simulink model "MMC_Per_arm_outer_v5_G2_case2_clip_delay1p4_aligned"  (R2024a)
settings: Solver=FixedStepDiscrete  StartTime=0.0  StopTime=2  FixedStep=Ts  RelTol=1e-3
PreLoadFcn:
  | % ---- MMC_Inner4 workspace parameters (control gains live inside the MATLAB Function blocks) ----
  | % ---------------- Converter ----------------
  | VDC     = 800;                  % DC-link voltage (V)  -> Vdc_pos / Vdc_neg = VDC/2
  | N       = 8;                    % submodules per arm
  | C       = 2.2e-3;               % submodule capacitance (F)  -> HB_xx blocks
  | vo      = 100;                  % nominal = initial capacitor voltage (V) = VDC/N  -> HB_xx, Vc_nom
  | W_nom   = 0.5*C*N*vo^2;         % nominal arm energy (J) -> initial condition of the Comm delay blocks
  | Larm    = 5e-3;                 % arm inductance (H)
  | Rarm    = 0.5;                  % arm resistance (ohm)
  | 
  | % ---------------- Grid and PCC filter ----------------
  | f       = 50;                   % grid frequency (Hz)
  | Vg_rms  = 230;                  % grid RMS voltage (V)
  | Vg_pk   = Vg_rms*sqrt(2);       % grid peak voltage (V) -> AC Voltage Source
  | Lg      = 2e-3;                 % line inductance (H)
  | Rg      = 0.1;                  % line resistance (ohm)
  | Cf      = 10e-6;                % AC filter capacitance (F)
  | Rf      = 10;                   % AC filter damping resistance (ohm)
  | 
  | % ---------------- Power set-points ----------------
  | Pstar   = 1500;                 % active-power set-point (W)
  | Qstar   = 0;                    % reactive-power set-point (var)
  | 
  | % ---------------- Timing ----------------
  | fsw     = 1250;                 % carrier frequency per submodule (Hz) -> N*fsw = 10 kHz per arm
  | Ts      = 1e-5;                 % simulation step = submodule-layer step (s)
  | Ts_ctrl = 1e-4;                 % arm-leader control step (s)
  | % ---------------- Test schedule: P* staircase and PCC load (added in _tests) ----------------
  | P_base   = 1500;                % staircase base = first level (W)
  | dP_step  = 250;                 % staircase step (W): 1500 -> 1750 -> 2000 -> 2250 -> 2500
  | t_step   = [0.6 1.0 1.4 1.8];   % step instants (s), 0.4 s hold at each level
  | t_back   = 2.2;                 % return to P_base (s) before the load test
  | P_load1  = 1000;                % PCC load 1 (W at 230 V rms)
  | P_load2  = 1000;                % PCC load 2 (W at 230 V rms)
  | R_load1  = Vg_rms^2/P_load1;    % 52.9 ohm
  | R_load2  = Vg_rms^2/P_load2;    % 52.9 ohm
  | t_load1  = 2.4;                 % Breaker load 1: closes at 2.4 s (stays closed)
  | t_load2  = [2.7 3.0];           % Breaker load 2: closes at 2.7 s, opens at 3.0 s
  | % ---- CASE: initial imbalance HB_u3 = 110 V, HB_u6 = 90 V, P* fixed 1500 W, no PCC load, 2 s
  | % ---- DERIVED: case2_clip_delay1p4_aligned: case 2 clip + time-aligned delay 140 samples (1.4 ms) -- eq. (6) test below the bound
  | % ---- DERIVED: case2_clip: same as case 2 + correction bounded to |k_v*err| <= 0.1 in hb_sm_local_ctrl (16 charts)
  | % P_SLEW = 5000 W/s, I_max = 17 A, P_max = 2500 W are set INSIDE mmc_outer_ctrl (both arm leaders)
  | t_load1  = 10;  t_load2 = [10 11];   % PCC load test disabled in this case (beyond StopTime)
  | Vc0_u3   = 110;                 % initial capacitor voltage of HB_u3 (V)
  | Vc0_u6   = 90;                  % initial capacitor voltage of HB_u6 (V)
InitFcn:
  | % ---- MMC_Inner4 workspace parameters (control gains live inside the MATLAB Function blocks) ----
  | % ---------------- Converter ----------------
  | VDC     = 800;                  % DC-link voltage (V)  -> Vdc_pos / Vdc_neg = VDC/2
  | N       = 8;                    % submodules per arm
  | C       = 2.2e-3;               % submodule capacitance (F)  -> HB_xx blocks
  | vo      = 100;                  % nominal = initial capacitor voltage (V) = VDC/N  -> HB_xx, Vc_nom
  | W_nom   = 0.5*C*N*vo^2;         % nominal arm energy (J) -> initial condition of the Comm delay blocks
  | Larm    = 5e-3;                 % arm inductance (H)
  | Rarm    = 0.5;                  % arm resistance (ohm)
  | 
  | % ---------------- Grid and PCC filter ----------------
  | f       = 50;                   % grid frequency (Hz)
  | Vg_rms  = 230;                  % grid RMS voltage (V)
  | Vg_pk   = Vg_rms*sqrt(2);       % grid peak voltage (V) -> AC Voltage Source
  | Lg      = 2e-3;                 % line inductance (H)
  | Rg      = 0.1;                  % line resistance (ohm)
  | Cf      = 10e-6;                % AC filter capacitance (F)
  | Rf      = 10;                   % AC filter damping resistance (ohm)
  | 
  | % ---------------- Power set-points ----------------
  | Pstar   = 1500;                 % active-power set-point (W)
  | Qstar   = 0;                    % reactive-power set-point (var)
  | 
  | % ---------------- Timing ----------------
  | fsw     = 1250;                 % carrier frequency per submodule (Hz) -> N*fsw = 10 kHz per arm
  | Ts      = 1e-5;                 % simulation step = submodule-layer step (s)
  | Ts_ctrl = 1e-4;                 % arm-leader control step (s)
  | % ---------------- Test schedule: P* staircase and PCC load (added in _tests) ----------------
  | P_base   = 1500;                % staircase base = first level (W)
  | dP_step  = 250;                 % staircase step (W): 1500 -> 1750 -> 2000 -> 2250 -> 2500
  | t_step   = [0.6 1.0 1.4 1.8];   % step instants (s), 0.4 s hold at each level
  | t_back   = 2.2;                 % return to P_base (s) before the load test
  | P_load1  = 1000;                % PCC load 1 (W at 230 V rms)
  | P_load2  = 1000;                % PCC load 2 (W at 230 V rms)
  | R_load1  = Vg_rms^2/P_load1;    % 52.9 ohm
  | R_load2  = Vg_rms^2/P_load2;    % 52.9 ohm
  | t_load1  = 2.4;                 % Breaker load 1: closes at 2.4 s (stays closed)
  | t_load2  = [2.7 3.0];           % Breaker load 2: closes at 2.7 s, opens at 3.0 s
  | % ---- CASE: initial imbalance HB_u3 = 110 V, HB_u6 = 90 V, P* fixed 1500 W, no PCC load, 2 s
  | % ---- DERIVED: case2_clip_delay1p4_aligned: case 2 clip + time-aligned delay 140 samples (1.4 ms) -- eq. (6) test below the bound
  | % ---- DERIVED: case2_clip: same as case 2 + correction bounded to |k_v*err| <= 0.1 in hb_sm_local_ctrl (16 charts)
  | % P_SLEW = 5000 W/s, I_max = 17 A, P_max = 2500 W are set INSIDE mmc_outer_ctrl (both arm leaders)
  | t_load1  = 10;  t_load2 = [10 11];   % PCC load test disabled in this case (beyond StopTime)
  | Vc0_u3   = 110;                 % initial capacitor voltage of HB_u3 (V)
  | Vc0_u6   = 90;                  % initial capacitor voltage of HB_u6 (V)
libraries: spsHalfBridgeMMCLib x16, spsSeriesRLCBranchLib x6, spsCurrentMeasurementLib x5, spsBreakerLib x2, spsGroundLib x2, spsDCVoltageSourceLib x2, spsACVoltageSourceLib x1, spspowerguiLib x1, spsVoltageMeasurementLib x1
(part 4 of 6)

== matlab function MMC_Per_arm_outer_v5_G2_case2_clip_delay1p4_aligned/SM_l7/Local Ctrl ==
  data: sm_id input; S_top output; m_arm input; i_arm input; Vc_i input; Vc_prev input; Vc_next input; t input; S_bot output
function [S_top, S_bot] = hb_sm_local_ctrl(sm_id, m_arm, i_arm, Vc_i, Vc_prev, Vc_next, t)
%#codegen
% =========================================================================
% HB_SM_LOCAL_CTRL  -  Submodule local controller: neighbour balancing + PSC-PWM
% -------------------------------------------------------------------------
% Block     : "Local Ctrl" inside every SM_ux / SM_lx subsystem
% Rate      : Ts = 10 us
% Instances : 16 (one per half-bridge submodule)
% Purpose   : decide the two gate signals of ONE half-bridge submodule using
%             only local information: own capacitor voltage, the two ring
%             neighbours, the arm modulation index sent by the arm leader,
%             the arm-current direction and the time base.
%             No sorting and no access to the full capacitor-voltage vector.
% Inputs    : sm_id    own index 1..N (sets the carrier phase shift)
%             m_arm    arm modulation index from the arm leader, in [0, 1]
%             i_arm    arm current (A), only its direction is used
%             Vc_i     own capacitor voltage (V)
%             Vc_prev  previous ring neighbour voltage (V)
%             Vc_next  next ring neighbour voltage (V)
%             t        simulation time (s), carrier time base
% Outputs   : S_top    upper switch gate (1 = on)  -> capacitor INSERTED (+Vc)
%             S_bot    lower switch gate (1 = on)  -> capacitor BYPASSED (0 V)
% =========================================================================

%% ---------------- PARAMETERS ----------------
N      = 8;                              % submodules per arm -> carrier phase shift of SM k = (k-1)/N of a period
fsw    = 1250;                           % carrier frequency per submodule (Hz) -> N*fsw = 10 kHz apparent arm ripple
k_v    = 0.2;                            % balancing gain (1/V): modulation-index change per volt of error
dead   = 0.1;                            % dead-band (V): errors smaller than this are ignored (no chattering)
Iscale = 1.0;                            % current scale (A) of the smooth sign function tanh(i_arm/Iscale)
dm_max = 0.1;                            % BOUND on the correction: |k_v*err| <= dm_max  (CLIP case, Delta d_max = 0.1)

%% ---------------- 1. neighbour-average balancing correction ----------------
err  = 0.5*(Vc_prev + Vc_next) - Vc_i;   % error = neighbour average - own voltage (> 0: I am too low, I need charging)
if abs(err) < dead                       % error inside the dead-band?
    err = 0;                             % ignore it
end
dirn = tanh(i_arm / Iscale);             % smooth current direction in (-1, +1); > 0 means inserting CHARGES the capacitor
c    = min(max(k_v * err, -dm_max), dm_max);   % bounded correction magnitude: |k_v e_i| <= dm_max (a 10 V error no longer saturates the duty)
dm   = c * dirn;                         % correction: insert more if charging is needed AND the current charges, less otherwise
m_i  = min(max(m_arm + dm, 0), 1);       % own modulation index = arm index + correction, clamped to [0, 1]

%% ---------------- 2. phase-shifted triangular carrier (0 -> 1 -> 0) ----------------
tau = mod(t*fsw + (sm_id - 1)/N, 1);     % position inside the carrier period, in [0, 1), shifted by (sm_id-1)/N
car = 1 - abs(2*tau - 1);                % triangle: rises 0 -> 1 on the first half, falls 1 -> 0 on the second half

%% ---------------- 3. half-bridge gating ----------------
if m_i >= car                            % modulation index above the carrier?
    S_top = 1;                           % upper switch on  -> capacitor inserted (+Vc on the arm)
    S_bot = 0;                           % lower switch off
else                                     % modulation index below the carrier
    S_top = 0;                           % upper switch off
    S_bot = 1;                           % lower switch on  -> capacitor bypassed (0 V)
end
end

== matlab function MMC_Per_arm_outer_v5_G2_case2_clip_delay1p4_aligned/SM_u8/Neighbors ==
  data: Vc_arm input; Vc_i output; i input; Vc_prev output; Vc_next output
function [Vc_i, Vc_prev, Vc_next] = get_neighbors(Vc_arm, i)
%#codegen
% =========================================================================
% GET_NEIGHBORS  -  Ring-link emulation for submodule number i
% -------------------------------------------------------------------------
% Block     : "Neighbors" inside every SM_ux / SM_lx subsystem
% Rate      : Ts = 10 us
% Instances : 16 (one per submodule)
% Purpose   : in simulation the whole capacitor-voltage vector of the arm is
%             available, but a real submodule only knows its OWN voltage and
%             the voltages of its two ring neighbours. This block hides
%             everything else, so the local controller stays truly local.
% Inputs    : Vc_arm  N x 1 vector of capacitor voltages of the arm (V)
%             i       own submodule index, 1..N
% Outputs   : Vc_i    own capacitor voltage (V)
%             Vc_prev voltage of the previous ring neighbour (V)
%             Vc_next voltage of the next ring neighbour (V)
% =========================================================================

%% ---------------- PARAMETERS ----------------
N = 8;                                   % submodules per arm (= length of Vc_arm, the Mux of the 8 HB voltages)
ND = 140;                             % ALIGNED-DELAY case: own AND neighbour values delayed by ND samples (Ts = 10 us -> 1.4 ms)
persistent buf_i buf_p buf_n idx         % circular buffers of the own sample and the two neighbour links, and the index

%% ---------------- 1. own index, made safe ----------------
k = min(max(round(i), 1), N);            % round to an integer and clamp to [1, N] (protects against a bad sm_id)

%% ---------------- 2. own voltage ----------------
Vc_i = Vc_arm(k);                        % own capacitor voltage

%% ---------------- 3. ring neighbours (circular: SM1 and SMN are neighbours) ----------------
if k == 1                                % first submodule of the ring
    Vc_prev = Vc_arm(N);                 % previous neighbour wraps around to the last submodule
    Vc_next = Vc_arm(2);                 % next neighbour is SM2
elseif k == N                            % last submodule of the ring
    Vc_prev = Vc_arm(N - 1);             % previous neighbour is SM(N-1)
    Vc_next = Vc_arm(1);                 % next neighbour wraps around to SM1
else                                     % any submodule in the middle
    Vc_prev = Vc_arm(k - 1);             % previous neighbour
    Vc_next = Vc_arm(k + 1);             % next neighbour
end

%% ---------------- 4. time-aligned delay: own sample and neighbour links delayed by the same ND (ALIGNED-DELAY case) ----------------
if isempty(buf_i)                        % first call
    buf_i = Vc_i    * ones(ND, 1);       % buffers start filled with the first values: no false error during the first ND samples
    buf_p = Vc_prev * ones(ND, 1);
    buf_n = Vc_next * ones(ND, 1);
    idx   = 1;
end
d_i    = buf_i(idx);                     % own voltage ND samples ago (same instant as the neighbour values)
d_prev = buf_p(idx);                     % value sent by the previous neighbour ND samples ago
d_next = buf_n(idx);                     % value sent by the next neighbour ND samples ago
buf_i(idx) = Vc_i;                       % store the fresh values in the slot just read
buf_p(idx) = Vc_prev;
buf_n(idx) = Vc_next;
idx = idx + 1;                           % advance the circular index
if idx > ND
    idx = 1;
end
Vc_i    = d_i;                           % the local controller compares three values of the SAME instant t - tau
Vc_prev = d_prev;
Vc_next = d_next;
end

== matlab function MMC_Per_arm_outer_v5_G2_case2_clip_delay1p4_aligned/SM_u8/Local Ctrl ==
  data: sm_id input; S_top output; m_arm input; i_arm input; Vc_i input; Vc_prev input; Vc_next input; t input; S_bot output
function [S_top, S_bot] = hb_sm_local_ctrl(sm_id, m_arm, i_arm, Vc_i, Vc_prev, Vc_next, t)
%#codegen
% =========================================================================
% HB_SM_LOCAL_CTRL  -  Submodule local controller: neighbour balancing + PSC-PWM
% -------------------------------------------------------------------------
% Block     : "Local Ctrl" inside every SM_ux / SM_lx subsystem
% Rate      : Ts = 10 us
% Instances : 16 (one per half-bridge submodule)
% Purpose   : decide the two gate signals of ONE half-bridge submodule using
%             only local information: own capacitor voltage, the two ring
%             neighbours, the arm modulation index sent by the arm leader,
%             the arm-current direction and the time base.
%             No sorting and no access to the full capacitor-voltage vector.
% Inputs    : sm_id    own index 1..N (sets the carrier phase shift)
%             m_arm    arm modulation index from the arm leader, in [0, 1]
%             i_arm    arm current (A), only its direction is used
%             Vc_i     own capacitor voltage (V)
%             Vc_prev  previous ring neighbour voltage (V)
%             Vc_next  next ring neighbour voltage (V)
%             t        simulation time (s), carrier time base
% Outputs   : S_top    upper switch gate (1 = on)  -> capacitor INSERTED (+Vc)
%             S_bot    lower switch gate (1 = on)  -> capacitor BYPASSED (0 V)
% =========================================================================

%% ---------------- PARAMETERS ----------------
N      = 8;                              % submodules per arm -> carrier phase shift of SM k = (k-1)/N of a period
fsw    = 1250;                           % carrier frequency per submodule (Hz) -> N*fsw = 10 kHz apparent arm ripple
k_v    = 0.2;                            % balancing gain (1/V): modulation-index change per volt of error
dead   = 0.1;                            % dead-band (V): errors smaller than this are ignored (no chattering)
Iscale = 1.0;                            % current scale (A) of the smooth sign function tanh(i_arm/Iscale)
dm_max = 0.1;                            % BOUND on the correction: |k_v*err| <= dm_max  (CLIP case, Delta d_max = 0.1)

%% ---------------- 1. neighbour-average balancing correction ----------------
err  = 0.5*(Vc_prev + Vc_next) - Vc_i;   % error = neighbour average - own voltage (> 0: I am too low, I need charging)
if abs(err) < dead                       % error inside the dead-band?
    err = 0;                             % ignore it
end
dirn = tanh(i_arm / Iscale);             % smooth current direction in (-1, +1); > 0 means inserting CHARGES the capacitor
c    = min(max(k_v * err, -dm_max), dm_max);   % bounded correction magnitude: |k_v e_i| <= dm_max (a 10 V error no longer saturates the duty)
dm   = c * dirn;                         % correction: insert more if charging is needed AND the current charges, less otherwise
m_i  = min(max(m_arm + dm, 0), 1);       % own modulation index = arm index + correction, clamped to [0, 1]

%% ---------------- 2. phase-shifted triangular carrier (0 -> 1 -> 0) ----------------
tau = mod(t*fsw + (sm_id - 1)/N, 1);     % position inside the carrier period, in [0, 1), shifted by (sm_id-1)/N
car = 1 - abs(2*tau - 1);                % triangle: rises 0 -> 1 on the first half, falls 1 -> 0 on the second half

%% ---------------- 3. half-bridge gating ----------------
if m_i >= car                            % modulation index above the carrier?
    S_top = 1;                           % upper switch on  -> capacitor inserted (+Vc on the arm)
    S_bot = 0;                           % lower switch off
else                                     % modulation index below the carrier
    S_top = 0;                           % upper switch off
    S_bot = 1;                           % lower switch on  -> capacitor bypassed (0 V)
end
end

== matlab function MMC_Per_arm_outer_v5_G2_case2_clip_delay1p4_aligned/SM_l8/Neighbors ==
  data: Vc_arm input; Vc_i output; i input; Vc_prev output; Vc_next output
function [Vc_i, Vc_prev, Vc_next] = get_neighbors(Vc_arm, i)
%#codegen
% =========================================================================
% GET_NEIGHBORS  -  Ring-link emulation for submodule number i
% -------------------------------------------------------------------------
% Block     : "Neighbors" inside every SM_ux / SM_lx subsystem
% Rate      : Ts = 10 us
% Instances : 16 (one per submodule)
% Purpose   : in simulation the whole capacitor-voltage vector of the arm is
%             available, but a real submodule only knows its OWN voltage and
%             the voltages of its two ring neighbours. This block hides
%             everything else, so the local controller stays truly local.
% Inputs    : Vc_arm  N x 1 vector of capacitor voltages of the arm (V)
%             i       own submodule index, 1..N
% Outputs   : Vc_i    own capacitor voltage (V)
%             Vc_prev voltage of the previous ring neighbour (V)
%             Vc_next voltage of the next ring neighbour (V)
% =========================================================================

%% ---------------- PARAMETERS ----------------
N = 8;                                   % submodules per arm (= length of Vc_arm, the Mux of the 8 HB voltages)
ND = 140;                             % ALIGNED-DELAY case: own AND neighbour values delayed by ND samples (Ts = 10 us -> 1.4 ms)
persistent buf_i buf_p buf_n idx         % circular buffers of the own sample and the two neighbour links, and the index

%% ---------------- 1. own index, made safe ----------------
k = min(max(round(i), 1), N);            % round to an integer and clamp to [1, N] (protects against a bad sm_id)

%% ---------------- 2. own voltage ----------------
Vc_i = Vc_arm(k);                        % own capacitor voltage

%% ---------------- 3. ring neighbours (circular: SM1 and SMN are neighbours) ----------------
if k == 1                                % first submodule of the ring
    Vc_prev = Vc_arm(N);                 % previous neighbour wraps around to the last submodule
    Vc_next = Vc_arm(2);                 % next neighbour is SM2
elseif k == N                            % last submodule of the ring
    Vc_prev = Vc_arm(N - 1);             % previous neighbour is SM(N-1)
    Vc_next = Vc_arm(1);                 % next neighbour wraps around to SM1
else                                     % any submodule in the middle
    Vc_prev = Vc_arm(k - 1);             % previous neighbour
    Vc_next = Vc_arm(k + 1);             % next neighbour
end

%% ---------------- 4. time-aligned delay: own sample and neighbour links delayed by the same ND (ALIGNED-DELAY case) ----------------
if isempty(buf_i)                        % first call
    buf_i = Vc_i    * ones(ND, 1);       % buffers start filled with the first values: no false error during the first ND samples
    buf_p = Vc_prev * ones(ND, 1);
    buf_n = Vc_next * ones(ND, 1);
    idx   = 1;
end
d_i    = buf_i(idx);                     % own voltage ND samples ago (same instant as the neighbour values)
d_prev = buf_p(idx);                     % value sent by the previous neighbour ND samples ago
d_next = buf_n(idx);                     % value sent by the next neighbour ND samples ago
buf_i(idx) = Vc_i;                       % store the fresh values in the slot just read
buf_p(idx) = Vc_prev;
buf_n(idx) = Vc_next;
idx = idx + 1;                           % advance the circular index
if idx > ND
    idx = 1;
end
Vc_i    = d_i;                           % the local controller compares three values of the SAME instant t - tau
Vc_prev = d_prev;
Vc_next = d_next;
end

== matlab function MMC_Per_arm_outer_v5_G2_case2_clip_delay1p4_aligned/SM_l8/Local Ctrl ==
  data: sm_id input; S_top output; m_arm input; i_arm input; Vc_i input; Vc_prev input; Vc_next input; t input; S_bot output
function [S_top, S_bot] = hb_sm_local_ctrl(sm_id, m_arm, i_arm, Vc_i, Vc_prev, Vc_next, t)
%#codegen
% =========================================================================
% HB_SM_LOCAL_CTRL  -  Submodule local controller: neighbour balancing + PSC-PWM
% -------------------------------------------------------------------------
% Block     : "Local Ctrl" inside every SM_ux / SM_lx subsystem
% Rate      : Ts = 10 us
% Instances : 16 (one per half-bridge submodule)
% Purpose   : decide the two gate signals of ONE half-bridge submodule using
%             only local information: own capacitor voltage, the two ring
%             neighbours, the arm modulation index sent by the arm leader,
%             the arm-current direction and the time base.
%             No sorting and no access to the full capacitor-voltage vector.
% Inputs    : sm_id    own index 1..N (sets the carrier phase shift)
%             m_arm    arm modulation index from the arm leader, in [0, 1]
%             i_arm    arm current (A), only its direction is used
%             Vc_i     own capacitor voltage (V)
%             Vc_prev  previous ring neighbour voltage (V)
%             Vc_next  next ring neighbour voltage (V)
%             t        simulation time (s), carrier time base
% Outputs   : S_top    upper switch gate (1 = on)  -> capacitor INSERTED (+Vc)
%             S_bot    lower switch gate (1 = on)  -> capacitor BYPASSED (0 V)
% =========================================================================

%% ---------------- PARAMETERS ----------------
N      = 8;                              % submodules per arm -> carrier phase shift of SM k = (k-1)/N of a period
fsw    = 1250;                           % carrier frequency per submodule (Hz) -> N*fsw = 10 kHz apparent arm ripple
k_v    = 0.2;                            % balancing gain (1/V): modulation-index change per volt of error
dead   = 0.1;                            % dead-band (V): errors smaller than this are ignored (no chattering)
Iscale = 1.0;                            % current scale (A) of the smooth sign function tanh(i_arm/Iscale)
dm_max = 0.1;                            % BOUND on the correction: |k_v*err| <= dm_max  (CLIP case, Delta d_max = 0.1)

%% ---------------- 1. neighbour-average balancing correction ----------------
err  = 0.5*(Vc_prev + Vc_next) - Vc_i;   % error = neighbour average - own voltage (> 0: I am too low, I need charging)
if abs(err) < dead                       % error inside the dead-band?
    err = 0;                             % ignore it
end
dirn = tanh(i_arm / Iscale);             % smooth current direction in (-1, +1); > 0 means inserting CHARGES the capacitor
c    = min(max(k_v * err, -dm_max), dm_max);   % bounded correction magnitude: |k_v e_i| <= dm_max (a 10 V error no longer saturates the duty)
dm   = c * dirn;                         % correction: insert more if charging is needed AND the current charges, less otherwise
m_i  = min(max(m_arm + dm, 0), 1);       % own modulation index = arm index + correction, clamped to [0, 1]

%% ---------------- 2. phase-shifted triangular carrier (0 -> 1 -> 0) ----------------
tau = mod(t*fsw + (sm_id - 1)/N, 1);     % position inside the carrier period, in [0, 1), shifted by (sm_id-1)/N
car = 1 - abs(2*tau - 1);                % triangle: rises 0 -> 1 on the first half, falls 1 -> 0 on the second half

%% ---------------- 3. half-bridge gating ----------------
if m_i >= car                            % modulation index above the carrier?
    S_top = 1;                           % upper switch on  -> capacitor inserted (+Vc on the arm)
    S_bot = 0;                           % lower switch off
else                                     % modulation index below the carrier
    S_top = 0;                           % upper switch off
    S_bot = 1;                           % lower switch on  -> capacitor bypassed (0 V)
end
end

== matlab function MMC_Per_arm_outer_v5_G2_case2_clip_delay1p4_aligned/Meas Filter MA10 ==
  data: v_ac input; v_ac_f output; i_ac input; i_u input; i_l input; i_ac_f output; i_u_f output; i_l_f output
function [v_ac_f, i_ac_f, i_u_f, i_l_f] = meas_avg(v_ac, i_ac, i_u, i_l)
%#codegen
% =========================================================================
% MEAS_AVG  -  Measurement filter: 10-sample moving average
% -------------------------------------------------------------------------
% Block     : "Meas Filter MA10" (root level)
% Rate      : Ts = 10 us (switching-layer rate)
% Instances : 1
% Purpose   : average the last 10 samples (= one period of the 10 kHz PWM
%             ripple) so the ripple is removed BEFORE the Rate Transition
%             blocks slow the signals down to Ts_ctrl = 100 us (no aliasing).
% Inputs    : v_ac  PCC voltage (V)        i_ac  grid current (A)
%             i_u   upper-arm current (A)  i_l   lower-arm current (A)
% Outputs   : the same four signals, filtered
% =========================================================================

%% ---------------- PARAMETERS ----------------
M = 10;                                  % window length (samples): 10 x 10 us = 100 us = one 10 kHz ripple period

%% ---------------- PERSISTENT STATES ----------------
persistent buf idx                       % buf: last M samples (M x 4 matrix); idx: next row to overwrite
if isempty(buf)                          % first call only
    buf = zeros(M, 4);                   % start with an all-zero window
    idx = 1;                             % write pointer on row 1
end

%% ---------------- 1. store the new samples ----------------
buf(idx, :) = [v_ac, i_ac, i_u, i_l];   % overwrite the oldest row with the four new samples
idx = idx + 1;                           % move the write pointer forward
if idx > M                               % past the last row?
    idx = 1;                             % wrap around (circular buffer)
end

%% ---------------- 2. average over the window ----------------
y = sum(buf, 1) / M;                     % column-wise mean -> 1 x 4 vector of averages

%% ---------------- 3. outputs ----------------
v_ac_f = y(1);                           % filtered PCC voltage
i_ac_f = y(2);                           % filtered grid current
i_u_f  = y(3);                           % filtered upper-arm current
i_l_f  = y(4);                           % filtered lower-arm current
end

== matlab function MMC_Per_arm_outer_v5_G2_case2_clip_delay1p4_aligned/SM_l1/Neighbors ==
  data: Vc_arm input; Vc_i output; i input; Vc_prev output; Vc_next output
function [Vc_i, Vc_prev, Vc_next] = get_neighbors(Vc_arm, i)
%#codegen
% =========================================================================
% GET_NEIGHBORS  -  Ring-link emulation for submodule number i
% -------------------------------------------------------------------------
% Block     : "Neighbors" inside every SM_ux / SM_lx subsystem
% Rate      : Ts = 10 us
% Instances : 16 (one per submodule)
% Purpose   : in simulation the whole capacitor-voltage vector of the arm is
%             available, but a real submodule only knows its OWN voltage and
%             the voltages of its two ring neighbours. This block hides
%             everything else, so the local controller stays truly local.
% Inputs    : Vc_arm  N x 1 vector of capacitor voltages of the arm (V)
%             i       own submodule index, 1..N
% Outputs   : Vc_i    own capacitor voltage (V)
%             Vc_prev voltage of the previous ring neighbour (V)
%             Vc_next voltage of the next ring neighbour (V)
% =========================================================================

%% ---------------- PARAMETERS ----------------
N = 8;                                   % submodules per arm (= length of Vc_arm, the Mux of the 8 HB voltages)
ND = 140;                             % ALIGNED-DELAY case: own AND neighbour values delayed by ND samples (Ts = 10 us -> 1.4 ms)
persistent buf_i buf_p buf_n idx         % circular buffers of the own sample and the two neighbour links, and the index

%% ---------------- 1. own index, made safe ----------------
k = min(max(round(i), 1), N);            % round to an integer and clamp to [1, N] (protects against a bad sm_id)

%% ---------------- 2. own voltage ----------------
Vc_i = Vc_arm(k);                        % own capacitor voltage

%% ---------------- 3. ring neighbours (circular: SM1 and SMN are neighbours) ----------------
if k == 1                                % first submodule of the ring
    Vc_prev = Vc_arm(N);                 % previous neighbour wraps around to the last submodule
    Vc_next = Vc_arm(2);                 % next neighbour is SM2
elseif k == N                            % last submodule of the ring
    Vc_prev = Vc_arm(N - 1);             % previous neighbour is SM(N-1)
    Vc_next = Vc_arm(1);                 % next neighbour wraps around to SM1
else                                     % any submodule in the middle
    Vc_prev = Vc_arm(k - 1);             % previous neighbour
    Vc_next = Vc_arm(k + 1);             % next neighbour
end

%% ---------------- 4. time-aligned delay: own sample and neighbour links delayed by the same ND (ALIGNED-DELAY case) ----------------
if isempty(buf_i)                        % first call
    buf_i = Vc_i    * ones(ND, 1);       % buffers start filled with the first values: no false error during the first ND samples
    buf_p = Vc_prev * ones(ND, 1);
    buf_n = Vc_next * ones(ND, 1);
    idx   = 1;
end
d_i    = buf_i(idx);                     % own voltage ND samples ago (same instant as the neighbour values)
d_prev = buf_p(idx);                     % value sent by the previous neighbour ND samples ago
d_next = buf_n(idx);                     % value sent by the next neighbour ND samples ago
buf_i(idx) = Vc_i;                       % store the fresh values in the slot just read
buf_p(idx) = Vc_prev;
buf_n(idx) = Vc_next;
idx = idx + 1;                           % advance the circular index
if idx > ND
    idx = 1;
end
Vc_i    = d_i;                           % the local controller compares three values of the SAME instant t - tau
Vc_prev = d_prev;
Vc_next = d_next;
end

== matlab function MMC_Per_arm_outer_v5_G2_case2_clip_delay1p4_aligned/Arm Leader UPPER/Outer Loop ==
  data: v_ac input; i_ac_ref output; i_ac input; Pstar input; Qstar input; t input; theta output; V_amp output; P_meas output; Q_meas output
function [i_ac_ref, theta, V_amp, P_meas, Q_meas] = mmc_outer_ctrl(v_ac, i_ac, Pstar, Qstar, t)
%#codegen
% =========================================================================
% MMC_OUTER_CTRL  -  Outer loop: grid synchronisation (SOGI-PLL) + P/Q control
% -------------------------------------------------------------------------
% Block     : "Outer Loop" inside Arm Leader UPPER and Arm Leader LOWER
% Rate      : Ts_ctrl = 100 us
% Instances : 2 (one per arm leader)
% Purpose   : build the grid-current reference i_ac_ref from the power
%             set-points. Both arm leaders run this identical code on the
%             same measurements, so they obtain the SAME i_ac_ref without
%             exchanging any data.
%   1. SOGI on v_ac and i_ac   -> orthogonal (alpha, beta) components
%   2. SOGI-PLL                -> theta locked on v_ac  (v_alpha = V_amp*cos(theta))
%   3. P = 0.5*(va*ia + vb*ib),  Q = 0.5*(va*ib - vb*ia)   (Q > 0: current LEADS voltage)
%   4. P/Q PI loops + feed-forward -> current components Ip, Iq
%   5. i_ac_ref = Ip*cos(theta) - Iq*sin(theta)
% Inputs    : v_ac   PCC voltage (V)          i_ac   grid current (A)
%             Pstar  active-power set-point (W)   Qstar  reactive-power set-point (var)
%             t      simulation time (s), used for the soft start
% Outputs   : i_ac_ref (A), theta (rad), V_amp (V), P_meas (W), Q_meas (var)
% =========================================================================

%% ---------------- PARAMETERS: timing and grid ----------------
Ts      = 1e-4;                          % execution period (s) = Ts_ctrl
f0      = 50;                            % grid frequency (Hz)
w0      = 2*pi*f0;                       % grid angular frequency (rad/s)
USE_PLL = true;                          % true: PLL locked on v_ac (grid-connected); false: free-running 50 Hz angle (standalone tests)
NMA     = 200;                           % moving-average length for P and Q: 200 x 100 us = 20 ms = one grid period

%% ---------------- PARAMETERS: soft start ----------------
T_START = 0.15;                          % (s) references held at zero until the PLL has locked
PQ_RAMP = 10000;                         % (W/s and var/s) reference ramp rate after T_START
P_SLEW  = 5000;                          % (W/s) slew-rate limit on the external set-point Pstar (a 250 W step is ramped over 50 ms)

%% ---------------- PARAMETERS: SOGI and PLL ----------------
k_sogi = 1.41;                           % SOGI gain -> bandwidth ~ k*f0/2 = 35 Hz
Kp_pll = 50;                             % PLL proportional gain (rad/s per p.u. of vq)
Ki_pll = 1000;                           % PLL integral gain -> wn = 32 rad/s (5 Hz), zeta = 0.79
dw_max = 2*pi*5;                         % PLL integrator limit (rad/s) = +/- 5 Hz around f0
V_min  = 20;                             % (V) lower bound of the measured amplitude (division guard)
V_init = 300;                            % (V) initial amplitude estimate (close to the 325 V grid peak)
tau_v  = 0.01;                           % (s) low-pass time constant on the amplitude

%% ---------------- PARAMETERS: P and Q loops ----------------
% plant: P = 0.5*V_amp*Ip  ~ 163 W/A at 325 V  ->  closed-loop bandwidth ~ 5 Hz
Kp_pq = 0.004;                           % proportional gain (A/W)
Ki_pq = 0.2;                             % integral gain (A/(W*s))
I_max = 17;                              % (A) amplitude limit of each current component Ip, Iq (2500 W needs 15.4 A, +10 % for the PI)
P_max = 2500;                            % (W)   active-power reference limit (modulation headroom: m ~ 0.96 at 2500 W)
Q_max = 2000;                            % (var) reactive-power reference limit

%% ---------------- PERSISTENT STATES ----------------
persistent th pll_i v_alpha v_beta i_alpha i_beta Vf bufP bufQ idx xi_p xi_q P_lim
if isempty(th)                           % first call only
    th      = 0;                         % PLL angle (rad)
    pll_i   = 0;                         % PLL integrator (rad/s)
    v_alpha = 0;                         % SOGI in-phase state of the voltage (V)
    v_beta  = 0;                         % SOGI quadrature state of the voltage (V)
    i_alpha = 0;                         % SOGI in-phase state of the current (A)
    i_beta  = 0;                         % SOGI quadrature state of the current (A)
    Vf      = V_init;                    % filtered voltage amplitude (V)
    bufP    = zeros(NMA, 1);             % circular buffer of instantaneous P (W)
    bufQ    = zeros(NMA, 1);             % circular buffer of instantaneous Q (var)
    idx     = 1;                         % buffer write pointer
    xi_p    = 0;                         % integrator of the P loop (A)
    xi_q    = 0;                         % integrator of the Q loop (A)
    P_lim   = Pstar;                     % slew-limited P set-point (W), starts at the current set-point
end

%% ---------------- 1. SOGI filters (symplectic Euler: unity gain at w0) ----------------
v_alpha = v_alpha + Ts*(k_sogi*w0*(v_ac - v_alpha) - w0*v_beta);   % in-phase voltage component, band-passed at f0
v_beta  = v_beta  + Ts*w0*v_alpha;                                 % quadrature voltage component (lags by 90 deg)
i_alpha = i_alpha + Ts*(k_sogi*w0*(i_ac - i_alpha) - w0*i_beta);   % in-phase current component
i_beta  = i_beta  + Ts*w0*i_alpha;                                 % quadrature current component

%% ---------------- 2. voltage amplitude and PLL angle ----------------
Vn    = max(sqrt(v_alpha^2 + v_beta^2), V_min);                    % instantaneous amplitude, floored at V_min
Vf    = Vf + (Ts/(tau_v + Ts))*(Vn - Vf);                          % first-order low-pass filter (tau_v)
V_amp = Vf;                                                        % output: filtered amplitude
if USE_PLL                                                         % grid-connected mode
    vq    = (-sin(th)*v_alpha + cos(th)*v_beta)/Vn;                % normalised q-axis error (p.u.); zero when th is right
    pll_i = min(max(pll_i + Ki_pll*Ts*vq, -dw_max), dw_max);       % PI integrator, clamped to +/- dw_max
    th    = mod(th + (w0 + Kp_pll*vq + pll_i)*Ts, 2*pi);           % integrate the frequency, wrap to [0, 2*pi)
else                                                               % standalone mode
    th    = mod(w0*t, 2*pi);                                       % free-running angle at exactly f0
end
theta = th;                                                        % output: grid angle

%% ---------------- 3. measured P and Q (instantaneous, then 20 ms average) ----------------
bufP(idx) = 0.5*(v_alpha*i_alpha + v_beta*i_beta);                 % instantaneous active power (0.5: amplitudes, not RMS)
bufQ(idx) = 0.5*(v_alpha*i_beta  - v_beta*i_alpha);                % instantaneous reactive power (> 0: current leads)
idx = idx + 1;                                                     % advance the write pointer
if idx > NMA                                                       % past the end of the buffer?
    idx = 1;                                                       % wrap around
end
P_meas = sum(bufP)/NMA;                                            % 20 ms average -> removes 50 / 100 Hz residuals
Q_meas = sum(bufQ)/NMA;                                            % same for Q

%% ---------------- 4a. slew-rate limit on the external P set-point ----------------
P_lim = P_lim + min(max(Pstar - P_lim, -P_SLEW*Ts), P_SLEW*Ts);   % move P_lim towards Pstar by at most P_SLEW*Ts per step

%% ---------------- 4. soft-started references ----------------
if t < T_START                                                     % before the PLL has locked
    P_use = 0;                                                     % no active-power reference yet
    Q_use = 0;                                                     % no reactive-power reference yet
else                                                               % after T_START
    lim   = PQ_RAMP*(t - T_START);                                 % ramp envelope, grows linearly with time
    P_use = min(max(P_lim, -P_max), P_max);                        % clamp the (slew-limited) set-point to +/- P_max
    P_use = min(max(P_use, -lim),   lim);                          % then clamp it to the ramp envelope
    Q_use = min(max(Qstar, -Q_max), Q_max);                        % same for Q with +/- Q_max
    Q_use = min(max(Q_use, -lim),   lim);                          % and the same ramp envelope
end

%% ---------------- 5. P and Q loops -> current components (feed-forward + PI, clamping anti-windup) ----------------
Ip_ff = 2*P_use/V_amp;                                             % feed-forward: P = 0.5*V*I  ->  I = 2P/V
Iq_ff = 2*Q_use/V_amp;                                             % same for Q
e_p   = P_use - P_meas;                                            % active-power error (W)
e_q   = Q_use - Q_meas;                                            % reactive-power error (var)
Ip_un = Ip_ff + Kp_pq*e_p + xi_p;                                  % unsaturated active current (A)
if abs(Ip_un) < I_max                                              % integrate only when NOT saturated (anti-windup)
    xi_p = min(max(xi_p + Ki_pq*Ts*e_p, -I_max), I_max);           % integrator update, clamped
end
Iq_un = Iq_ff + Kp_pq*e_q + xi_q;                                  % unsaturated reactive current (A)
if abs(Iq_un) < I_max                                              % same anti-windup rule
    xi_q = min(max(xi_q + Ki_pq*Ts*e_q, -I_max), I_max);           % integrator update, clamped
end
Ip = min(max(Ip_un, -I_max), I_max);                               % final clamp of the active current
Iq = min(max(Iq_un, -I_max), I_max);                               % final clamp of the reactive current

%% ---------------- 6. AC current reference ----------------
i_ac_ref = Ip*cos(theta) - Iq*sin(theta);                          % in-phase (P) + quadrature (Q) components
end

== matlab function MMC_Per_arm_outer_v5_G2_case2_clip_delay1p4_aligned/Arm Leader UPPER/Inner Loop and Energy Balancing/B1 Arm Energy Estimation ==
  data: Vc_arm input; W_arm output; W_other input; Vc_nom input; Wo output; Wx output; W_nom output
function [W_arm, Wo, Wx, W_nom] = mmc_energy_estimation(Vc_arm, W_other, Vc_nom)
%#codegen
% =========================================================================
% MMC_ENERGY_ESTIMATION  -  Block B1: arm energy estimation and filtering
% -------------------------------------------------------------------------
% Block     : "B1 Arm Energy Estimation" inside Inner Loop and Energy Balancing
% Rate      : Ts_ctrl = 100 us
% Instances : 2 (one per arm leader)
% Purpose   : compute the energy stored in the own arm, average it and the
%             energy received from the other arm over one grid period, and
%             give the nominal arm energy used as the balancing target.
% Inputs    : Vc_arm   N x 1 capacitor voltages of the own arm (V)
%             W_other  raw energy received from the other arm leader (J)
%             Vc_nom   nominal capacitor voltage (V)
% Outputs   : W_arm    raw own energy (J)  -> sent to the other arm leader
%             Wo       filtered own energy (J)
%             Wx       filtered other-arm energy (J)
%             W_nom    nominal arm energy (J)
% =========================================================================

%% ---------------- PARAMETERS ----------------
C   = 2.2e-3;                            % submodule capacitance (F)
N   = 8;                                 % submodules per arm
NMA = 200;                               % moving-average length: 200 x 100 us = 20 ms = one grid period

%% ---------------- 1. nominal arm energy (balancing target) ----------------
W_nom = 0.5*C*N*Vc_nom^2;                % energy if all N capacitors sit exactly at Vc_nom

%% ---------------- PERSISTENT STATES ----------------
persistent bufO bufX idx                 % bufO: own-energy buffer; bufX: other-arm buffer; idx: write pointer
if isempty(idx)                          % first call only
    bufO = W_nom*ones(NMA, 1);           % pre-fill with the nominal energy (avoids a false start-up error)
    bufX = W_nom*ones(NMA, 1);           % same for the other arm
    idx  = 1;                            % write pointer on row 1
end

%% ---------------- 2. raw arm energy ----------------
W_arm = 0.5*C*sum(Vc_arm.^2);            % actual stored energy = sum over the N capacitors of 0.5*C*Vc^2

%% ---------------- 3. moving average of both energies ----------------
bufO(idx) = W_arm;                       % store the new own energy
bufX(idx) = W_other;                     % store the new other-arm energy
idx = idx + 1;                           % advance the write pointer
if idx > NMA                             % past the end of the buffer?
    idx = 1;                             % wrap around
end
Wo = sum(bufO)/NMA;                      % filtered own energy (50 / 100 Hz ripple removed)
Wx = sum(bufX)/NMA;                      % filtered other-arm energy
end
